simulink model "SteeringFull"  (R2025b)
settings: Solver=ode4  StartTime=0.0  StopTime=25  FixedStep=.001  RelTol=1e-3
undefined symbols (not defined in the file): dist_goal_ft, K_phi, K_rho, Kd_phi_out, Kp_phi_in, Kp_phi_out, Kp_rho_in, m2ft, N_filt, phi_goal_deg, phidot_max, rhodot_max, sigma_phi, sigma_rho, step_time, t_drive, V_bat, x0, y0
libraries: slpidlib x2
settings Model: Creator=jschw  LastModifiedBy=jschw

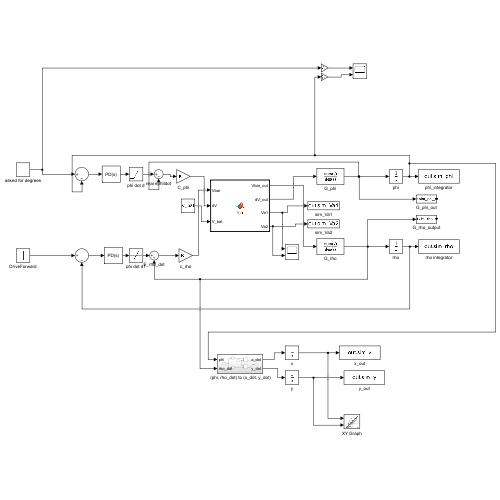
[thumbnail: Simulink's stored preview of the top-level diagram]
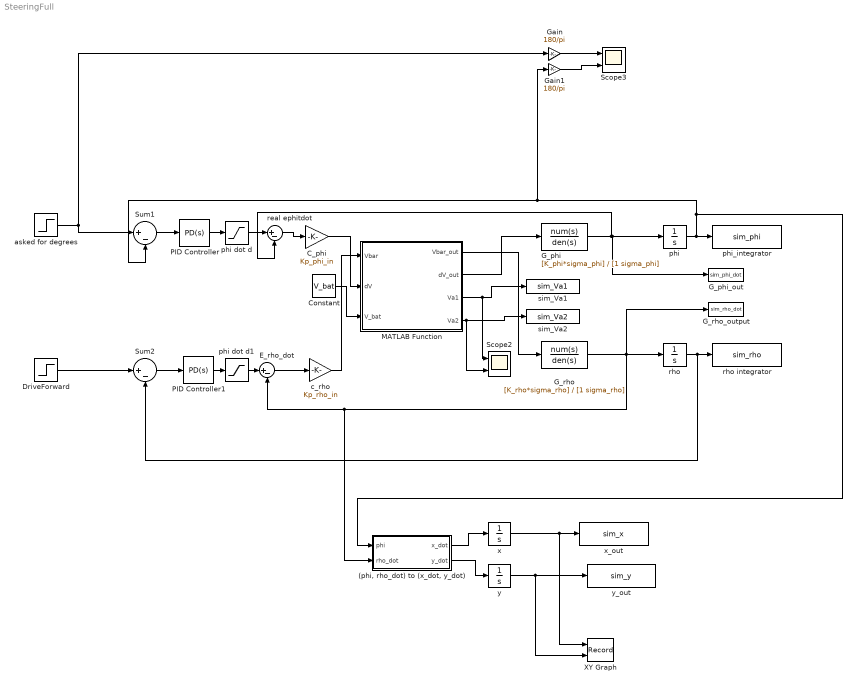
== system SteeringFull ==
  " (phi, rho_dot) to (x_dot, y_dot)" : Subsystem
  C_phi : Gain  Gain=Kp_phi_in
  Constant : Constant  Value=V_bat
  DriveForward : Step  Time=t_drive  After=dist_goal_ft/m2ft  SampleTime=0
  E_rho_dot : Sum  Inputs=|+-
  G_phi : TransferFcn  Numerator=[K_phi*sigma_phi]  Denominator=[1 sigma_phi]
  G_phi_out : ToWorkspace  VariableName=sim_phi_dot  SaveFormat=Timeseries  SampleTime=-1
  G_rho : TransferFcn  Numerator=[K_rho*sigma_rho]  Denominator=[1 sigma_rho]
  G_rho_output : ToWorkspace  VariableName=sim_rho_dot  SaveFormat=Timeseries  SampleTime=-1
  Gain : Gain  Gain=180/pi
  Gain1 : Gain  Gain=180/pi
  MATLAB Function : MATLAB Function  TreatAsAtomicUnit=on
  PID Controller : slpidlib/PID Controller  Controller=PD  Form=Parallel  TimeDomain=Continuous-time  UseExternalTs=off  SampleTime=-1  IntegratorMethod=Forward Euler  FilterMethod=Forward Euler  ControllerParametersSource=internal  P=Kp_phi_out  I=1  UseKiTs=off  D=Kd_phi_out  UseExternalDerivativeSource=off  N=N_filt  UseFilter=on  TunerSelectOption=Transfer Function Based (PID Tuner App)  InitialConditionSource=internal  InitialConditionForIntegrator=0  InitialConditionForFilter=0  DifferentiatorICPrevScaledInput=0  ExternalReset=none  TrackingMode=off  Kt=1  LimitOutput=off  SatLimitsSource=internal  UpperSaturationLimit=inf  LowerSaturationLimit=-inf  LinearizeAsGain=on  AntiWindupMode=none  Kb=1  LimitIntegrator=off  UpperIntegratorSaturationLimit=inf  LowerIntegratorSaturationLimit=-inf  POutMin=[]  POutMax=[]  IOutMin=[]  IOutMax=[]  DOutMin=[]  DOutMax=[]  NOutMin=[]  NOutMax=[]  SumOutMin=[]  SumOutMax=[]  SaturationOutMin=[]  SaturationOutMax=[]  PParamMin=[]  PParamMax=[]  IParamMin=[]  IParamMax=[]  DParamMin=[]  DParamMax=[]  NParamMin=[]  NParamMax=[]  KbParamMin=[]  KbParamMax=[]  KtParamMin=[]  KtParamMax=[]  KbOutMin=[]  KbOutMax=[]  KtOutMin=[]  KtOutMax=[]  IntegratorOutMin=[]  IntegratorOutMax=[]  FilterOutMin=[]  FilterOutMax=[]  SumI1OutMin=[]  SumI1OutMax=[]  SumI2OutMin=[]  SumI2OutMax=[]  SumI3OutMin=[]  SumI3OutMax=[]  SumI4OutMin=[]  SumI4OutMax=[]  SumDOutMin=[]  SumDOutMax=[]  DifferentiatorOutMin=[]  DifferentiatorOutMax=[]  FilterDiffOutCoefMin=[]  FilterDiffOutCoefMax=[]  ReciprocalOutMin=[]  ReciprocalOutMax=[]  SumDenOutMin=[]  SumDenOutMax=[]  SumNumOutMin=[]  SumNumOutMax=[]  DivideOutMin=[]  DivideOutMax=[]  UdiffTsProdOutMin=[]  UdiffTsProdOutMax=[]  NTsProdOutMin=[]  NTsProdOutMax=[]  UintegralTsProdOutMin=[]  UintegralTsProdOutMax=[]  UngainTsProdOutMin=[]  UngainTsProdOutMax=[]  ClampingZeroOutDataTypeStr=Inherit: Inherit via back propagation  ClampingZeroOutMin=[]  ClampingZeroOutMax=[]  FilterDenConstantOutDataTypeStr=Inherit: Inherit via back propagation  FilterDenConstantOutMin=[]  FilterDenConstantOutMax=[]  PCopyOutDataTypeStr=Inherit: Inherit via back propagation  PCopyOutMin=[]  PCopyOutMax=[]  NCopyOutDataTypeStr=Inherit: Inherit via back propagation  NCopyOutMin=[]  NCopyOutMax=[]  IntegratorContinuousStateAttributes=''  IntegratorStateMustResolveToSignalObject=off  IntegratorRTWStateStorageClass=Auto  FilterContinuousStateAttributes=''  FilterStateMustResolveToSignalObject=off  FilterRTWStateStorageClass=Auto  ParallelPVariant=InternalParameters  IdealPVariant=Disabled  IVariant=Disabled  DVariant=InternalParameters  IntegratorVariant=Disabled  SatVariant=Disabled  AWVariant=Disabled  PCopyVariant=Disabled  TRVariant=Disabled  FdbkBlocksVariant=Forward  IdealPFdbkVariant=Disabled  SatFdbkVariant=Disabled  DerivativeFilterVariant=ContFilter  NVariant=InternalParameters  NCopyVariant=Disabled  FilterICVariant=InternalICsFilter  IntegratorICVariant=Disabled  ExternalResetVariant=Disabled  TRSumVariant=Passthrough  SumFdbkVariant=Disabled  SumVariant=Sum_PD  TsampFilterVariant=InternalTs  TsampNgainVariant=Passthrough  TsampIntegralVariant=Disabled_SignalSpec  ExternalSaturationOutDataTypeStr=Inherit: Same as second input  DerivativeSourceVariant=ErrorSignal  PreIntVariant=InternalPreInt
  PID Controller1 : slpidlib/PID Controller  Controller=PD  Form=Parallel  TimeDomain=Continuous-time  UseExternalTs=off  SampleTime=-1  IntegratorMethod=Forward Euler  FilterMethod=Forward Euler  ControllerParametersSource=internal  P=Kp_phi_out  I=1  UseKiTs=off  D=Kd_phi_out  UseExternalDerivativeSource=off  N=N_filt  UseFilter=on  TunerSelectOption=Transfer Function Based (PID Tuner App)  InitialConditionSource=internal  InitialConditionForIntegrator=0  InitialConditionForFilter=0  DifferentiatorICPrevScaledInput=0  ExternalReset=none  TrackingMode=off  Kt=1  LimitOutput=off  SatLimitsSource=internal  UpperSaturationLimit=inf  LowerSaturationLimit=-inf  LinearizeAsGain=on  AntiWindupMode=none  Kb=1  LimitIntegrator=off  UpperIntegratorSaturationLimit=inf  LowerIntegratorSaturationLimit=-inf  POutMin=[]  POutMax=[]  IOutMin=[]  IOutMax=[]  DOutMin=[]  DOutMax=[]  NOutMin=[]  NOutMax=[]  SumOutMin=[]  SumOutMax=[]  SaturationOutMin=[]  SaturationOutMax=[]  PParamMin=[]  PParamMax=[]  IParamMin=[]  IParamMax=[]  DParamMin=[]  DParamMax=[]  NParamMin=[]  NParamMax=[]  KbParamMin=[]  KbParamMax=[]  KtParamMin=[]  KtParamMax=[]  KbOutMin=[]  KbOutMax=[]  KtOutMin=[]  KtOutMax=[]  IntegratorOutMin=[]  IntegratorOutMax=[]  FilterOutMin=[]  FilterOutMax=[]  SumI1OutMin=[]  SumI1OutMax=[]  SumI2OutMin=[]  SumI2OutMax=[]  SumI3OutMin=[]  SumI3OutMax=[]  SumI4OutMin=[]  SumI4OutMax=[]  SumDOutMin=[]  SumDOutMax=[]  DifferentiatorOutMin=[]  DifferentiatorOutMax=[]  FilterDiffOutCoefMin=[]  FilterDiffOutCoefMax=[]  ReciprocalOutMin=[]  ReciprocalOutMax=[]  SumDenOutMin=[]  SumDenOutMax=[]  SumNumOutMin=[]  SumNumOutMax=[]  DivideOutMin=[]  DivideOutMax=[]  UdiffTsProdOutMin=[]  UdiffTsProdOutMax=[]  NTsProdOutMin=[]  NTsProdOutMax=[]  UintegralTsProdOutMin=[]  UintegralTsProdOutMax=[]  UngainTsProdOutMin=[]  UngainTsProdOutMax=[]  ClampingZeroOutDataTypeStr=Inherit: Inherit via back propagation  ClampingZeroOutMin=[]  ClampingZeroOutMax=[]  FilterDenConstantOutDataTypeStr=Inherit: Inherit via back propagation  FilterDenConstantOutMin=[]  FilterDenConstantOutMax=[]  PCopyOutDataTypeStr=Inherit: Inherit via back propagation  PCopyOutMin=[]  PCopyOutMax=[]  NCopyOutDataTypeStr=Inherit: Inherit via back propagation  NCopyOutMin=[]  NCopyOutMax=[]  IntegratorContinuousStateAttributes=''  IntegratorStateMustResolveToSignalObject=off  IntegratorRTWStateStorageClass=Auto  FilterContinuousStateAttributes=''  FilterStateMustResolveToSignalObject=off  FilterRTWStateStorageClass=Auto  ParallelPVariant=InternalParameters  IdealPVariant=Disabled  IVariant=Disabled  DVariant=InternalParameters  IntegratorVariant=Disabled  SatVariant=Disabled  AWVariant=Disabled  PCopyVariant=Disabled  TRVariant=Disabled  FdbkBlocksVariant=Forward  IdealPFdbkVariant=Disabled  SatFdbkVariant=Disabled  DerivativeFilterVariant=ContFilter  NVariant=InternalParameters  NCopyVariant=Disabled  FilterICVariant=InternalICsFilter  IntegratorICVariant=Disabled  ExternalResetVariant=Disabled  TRSumVariant=Passthrough  SumFdbkVariant=Disabled  SumVariant=Sum_PD  TsampFilterVariant=InternalTs  TsampNgainVariant=Passthrough  TsampIntegralVariant=Disabled_SignalSpec  ExternalSaturationOutDataTypeStr=Inherit: Same as second input  DerivativeSourceVariant=ErrorSignal  PreIntVariant=InternalPreInt
  Scope2 : Scope  NumInputPorts=2
      settings: ActiveDisplayYMinimum=-12.221240321513863  ActiveDisplayYMaximum=13.778972051818078
  Scope3 : Scope  NumInputPorts=2
      settings: ActiveDisplayYMinimum=-45.362050824990007  ActiveDisplayYMaximum=-42.940666776961166
  Sum1 : Sum  Inputs=|+-
  Sum2 : Sum  Inputs=|+-
  XY Graph : Record  NumPorts=2.0  FileSettingsInternal="{\"entries\":[{\"content\":{\"excelSettings\":{\"content\":{},\"type\":\"Streamout.ExcelSettings\"},\"parquetSettings\":{\"content\":{},\"type\":\"Streamout.ParquetSettings\"}},\"type\":\"Streamout.FileSettingStorage\",\"uuid\":\"\"}],\"packageUris\":[\"http:\\/\\/schema.mathworks.com\\/mf0\\/streamout_blocks\\/R2020a\"],\"version\":\"1.0\"}"  FrameSettings=[0, 0]  Layout=[1 1]  SignalsInternal="{\"entries\":[{\"content\":{\"signals\":[{\"content\":{\"blockPath\":[],\"dimensions\":[1],\"domain\":\"\",\"lineColor\":\"#a2142f\",\"plots\":[ 1 ],\"port\":1,\"sid\":[\"\"],\"signalID\":1,\"signalName\":\"x\"},\"type\":\"RecordBlkView.Signal\",\"uuid\":\"\"},{\"content\":{\"blockPath\":[],\"dimensions\":[1],\"domain\":\"\",\"lineColor\":\"#139fff\",\"plots\":[ 1 ],\"port\":2,\"sid\":[\"\"],\"signalID\":2,\"signalName\":\"y\"},\"type\":\"RecordBlkView.Signal\",\"uuid\":\"\"}]},\"type\":\"RecordBlkView.InputSignals\",\"uuid\":\"\"}],\"packageUris\":[\"http:\\/\\/schema.mathworks.com\\/mf0\\/streamout_blocks\\/R2020a\"],\"version\":\"1.0\"}"  VisualizationBindings="{\"xyplotplugin\":{\"info\":[{\"series\":[{\"bindingParametersList\":[{\"parameter\":\"X-Axis\",\"signalID\":1,\"signalName\":\"x\"},{\"parameter\":\"Y-Axis\",\"signalID\":2,\"signalName\":\"y\"}],\"seriesID\":0}],\"subplotID\":1}]}}"  CompatibilityTag=XY
  asked for degrees : Step  Time=step_time  After=deg2rad(phi_goal_deg)  SampleTime=0
  c_rho : Gain  Gain=Kp_rho_in
  phi : Integrator
  phi dot d : Saturate  UpperLimit=phidot_max  LowerLimit=-phidot_max
  phi dot d1 : Saturate  UpperLimit=rhodot_max  LowerLimit=-rhodot_max
  phi_integrator : ToWorkspace  VariableName=sim_phi  SaveFormat=Timeseries  SampleTime=-1
  real ephitdot : Sum  Inputs=|+-
  rho : Integrator
  rho integrator : ToWorkspace  VariableName=sim_rho  SaveFormat=Timeseries  SampleTime=-1
  sim_Va1 : ToWorkspace  VariableName=sim_Va1  SaveFormat=Timeseries  SampleTime=-1
  sim_Va2 : ToWorkspace  VariableName=sim_Va2  SaveFormat=Timeseries  SampleTime=-1
  x : Integrator  InitialCondition=x0
  x_out : ToWorkspace  VariableName=sim_x  SaveFormat=Timeseries  SampleTime=-1
  y : Integrator  InitialCondition=y0
  y_out : ToWorkspace  VariableName=sim_y  SaveFormat=Timeseries  SampleTime=-1
  wires:
  E_rho_dot/1 -> c_rho/1
  c_rho/1 -> MATLAB Function/1(Vbar)
  Constant/1 -> MATLAB Function/3(V_bat)
  C_phi/1 -> MATLAB Function/2(dV)
  MATLAB Function/1(Vbar_out) -> G_rho/1
  MATLAB Function/2(dV_out) -> G_phi/1
  MATLAB Function/3(Va1) -> Scope2/1, sim_Va1/1
  MATLAB Function/4(Va2) -> Scope2/2, sim_Va2/1
  Sum1/1 -> PID Controller/1
  PID Controller/1 -> phi dot d/1
  phi dot d/1 -> real ephitdot/1
  asked for degrees/1 -> Sum1/1, Gain/1
  real ephitdot/1 -> C_phi/1
  G_phi/1 -> real ephitdot/2, G_phi_out/1, phi/1
  Gain1/1 -> Scope3/2
  Gain/1 -> Scope3/1
  Sum2/1 -> PID Controller1/1
  PID Controller1/1 -> phi dot d1/1
  phi dot d1/1 -> E_rho_dot/1
  DriveForward/1 -> Sum2/1
  rho/1 -> Sum2/2, rho integrator/1
  phi/1 -> " (phi, rho_dot) to (x_dot, y_dot)"/1(phi), Gain1/1, Sum1/2, phi_integrator/1
  G_rho/1 -> " (phi, rho_dot) to (x_dot, y_dot)"/2(rho_dot), E_rho_dot/2, G_rho_output/1, rho/1
  " (phi, rho_dot) to (x_dot, y_dot)"/2(y_dot) -> y/1
  " (phi, rho_dot) to (x_dot, y_dot)"/1(x_dot) -> x/1
  y/1 -> XY Graph/2, y_out/1
  x/1 -> XY Graph/1, x_out/1

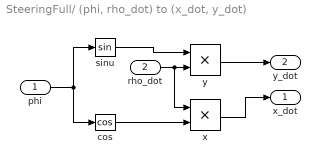
== system SteeringFull/ (phi, rho_dot) to (x_dot, y_dot) ==
  phi : Inport
  rho_dot : Inport  Port=2
  cos : Trigonometry  Operator=cos
  sinu : Trigonometry
  x : Product
  y : Product
  x_dot : Outport
  y_dot : Outport  Port=2
  wires:
  rho_dot/1 -> x/1, y/2
  phi/1 -> cos/1, sinu/1
  sinu/1 -> y/1
  cos/1 -> x/2
  x/1 -> x_dot/1
  y/1 -> y_dot/1

== matlab function SteeringFull/MATLAB Function ==
  data: Vbar input; Vbar_out output; dV input; V_bat input; dV_out output; Va1 output; Va2 output
function [Vbar_out, dV_out, Va1, Va2] = fcn(Vbar, dV, V_bat)
% Same saturation as SteeringInnerLoopTest.ino: scale both wheels
% together so the forward/turn ratio is kept
Va1 = (Vbar + dV)/2;
Va2 = (Vbar - dV)/2;
m = max(abs(Va1), abs(Va2));
if m > V_bat
    Va1 = Va1*V_bat/m;
    Va2 = Va2*V_bat/m;
end
Vbar_out = Va1 + Va2;
dV_out   = Va1 - Va2;
